simulink model "NexonEV_DriveCycle"  (R2026a)
settings: Solver=ode45  StopTime=360
settings Model: Creator=Prashanth  LastModifiedBy=Prashanth

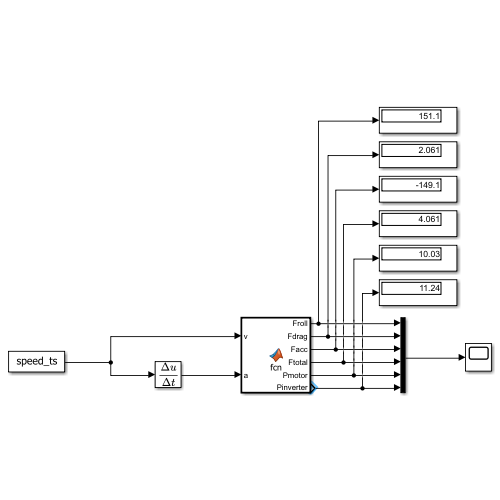
[thumbnail: Simulink's stored preview of the top-level diagram]
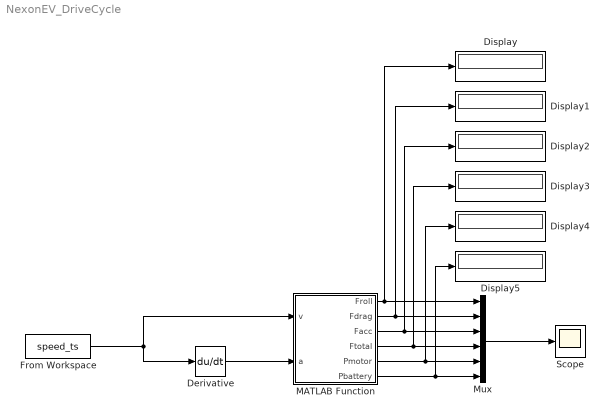
== system NexonEV_DriveCycle ==
  Derivative : Derivative
  Display{,1..5} (6 alike) : Display
  From Workspace : FromWorkspace  VariableName=speed_ts
  MATLAB Function : MATLAB Function  TreatAsAtomicUnit=on
  Mux : Mux  Inputs=6
  Scope : Scope
      settings: ActiveDisplayYMinimum=-2092.2116709094871  ActiveDisplayYMaximum=7000.6364482850513
  wires:
  Derivative/1 -> MATLAB Function/2(a)
  From Workspace/1 -> MATLAB Function/1(v), Derivative/1
  MATLAB Function/1(Froll) -> Display/1, Mux/1
  MATLAB Function/3(Facc) -> Display2/1, Mux/3
  MATLAB Function/2(Fdrag) -> Display1/1, Mux/2
  MATLAB Function/4(Ftotal) -> Display3/1, Mux/4
  MATLAB Function/5(Pmotor) -> Display4/1, Mux/5
  MATLAB Function/6(Pbattery) -> Display5/1, Mux/6
  Mux/1 -> Scope/1

== matlab function NexonEV_DriveCycle/MATLAB Function ==
  data: v input; Froll output; a input; Fdrag output; Facc output; Ftotal output; Pmotor output; Pbattery output

function [Froll, Fdrag, Facc, Ftotal, ...
          Pmotor, Pbattery] = fcn(v, a)

% Vehicle parameters
m = 1400;
g = 9.81;
Crr = 0.011;
Cd = 0.29;
A = 2.35;
rho = 1.225;

% Assumed efficiencies
eta_drive = 0.90;
eta_motor = 0.92;
eta_inv = 0.97;

% Rolling resistance force
Froll = Crr*m*g;

% Aerodynamic drag force
Fdrag = 0.5*rho*Cd*A*v^2;

% Acceleration force
Facc = m*a;

% Flat road assumption
Fgrade = 0;

% Total tractive force
Ftotal = Froll + Fdrag + Facc + Fgrade;

% Wheel mechanical power
Pwheel = Ftotal*v;

% Motor mechanical power, motoring only
Pmotor = max(Pwheel,0)/eta_drive;

% Inverter DC input power
Pbattery = Pmotor/(eta_motor*eta_inv);

end
